simulink model "a"  (Simulink 7.0)
settings: Solver=FixedStepDiscrete  StartTime=0.0  StopTime=10.0  FixedStep=0.001  RelTol=1e-3
libraries: dsPICdrivers x6, fuzblock x1
settings Model: Creator=Administrator  LastModifiedBy=Administrator
settings OptimizationCC: OptimizeModelRefInitCode=on  LifeSpan=1
settings HardwareCC: ProdBitPerInt=16  ProdEndianess=LittleEndian  ProdWordSize=16  ProdHWDeviceType=16-bit Generic
settings RTWCC: SystemTargetFile=dspic.tlc  TemplateMakefile=dspic_pic30_gcc.tmf  PostCodeGenCommand=dsPIC_Compile()  Description=Embedded Target for Microchip dsPIC (real-time)  ProcessScript=dspic_make_rtw_hook
settings CodeAppCC: IgnoreCustomStorageClasses=off
settings STFCustomTargetCC: GenFloatMathFcnCalls=ANSI_C  ModelReferenceCompliant=off  IncludeMdlTerminateFcn=off  CombineOutputUpdateFcns=on  SuppressErrorStatus=on  ERTCustomFileBanners=on  SupportContinuousTime=off  SupportNonInlinedSFcns=off  SystemTargetFile=dspic.tlc
settings ERTTargetCC: GenFloatMathFcnCalls=ANSI_C  ModelReferenceCompliant=off  CompOptLevelCompliant=off  IncludeMdlTerminateFcn=off  SuppressErrorStatus=on  ModelStepFunctionPrototypeControlCompliant=off  ExtModeMexFile=noextcomm  InlinedParameterPlacement=NonHierarchical  ERTSrcFileBannerTemplate=dsPIC_code_template.cgt  ERTHdrFileBannerTemplate=dsPIC_code_template.cgt  ERTDataSrcFileTemplate=dsPIC_code_template.cgt  ERTDataHdrFileTemplate=dsPIC_code_template.cgt  ERTCustomFileTemplate=dsPIC_main.tlc
settings CustomProperty: DataType=string  Value=C:\PROGRA~1\MATLAB\R2007b\bin\win32\gmake

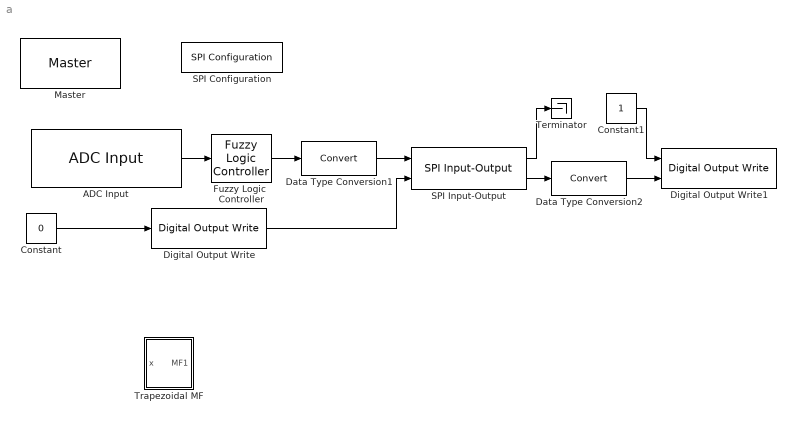
== system a ==
  ADC Input : dsPICdrivers/Peripheral I//O/ADC Input  Tag=dsPIC_ADC  Priority=5  ADC_TYPE=12 bits  ADC_MODE=Continuous sampling & get last channel value  NbrSampleStep=1  VoltRefpopup="AVdd  -  AVss"  OutFormatBitspopup=0000 dddd dddd dddd : Integer  InterruptPriority=6  ANCHANNELS=[8]  MaxName=ANmax = 4096  Rin=1e2  ADCS=6  SAMC=1  Temperature=25  DMAChannel=0  SampleTime=-1  Status="OK  |  Tsmp=7.000e-007 |  T/Channel=1.050e-005 |  Tall=1.050e-005"
  Constant : Constant  Value=0  OutDataTypeMode=boolean  OutDataType=sfix(16)  OutScaling=2^0
  Constant1 : Constant  OutDataTypeMode=boolean  OutDataType=sfix(16)  OutScaling=2^0
  Data Type Conversion1 : DataTypeConversion  OutDataTypeMode=uint16  OutDataType=sfix(16)  OutScaling=2^0
  Data Type Conversion2 : DataTypeConversion  OutDataTypeMode=boolean  OutDataType=sfix(16)  OutScaling=2^0
  Digital Output Write : dsPICdrivers/Digital I//O/Digital Output Write  Tag=dsPIC_Digital_Output  Priority=5  PORT=B  Pin=[2]  Simultaneous=off  OrderingInOutPopup=Output
  Digital Output Write1 : dsPICdrivers/Digital I//O/Digital Output Write  Tag=dsPIC_Digital_Output  Priority=5  PORT=B  Pin=[2]  Simultaneous=off  OrderingInOutPopup=Input
  Fuzzy Logic  Controller : fuzblock/Fuzzy Logic  Controller  SystemSampleTime=-1  fis=a1
  Master : dsPICdrivers/Master  Tag=dsPIC_MASTER  Priority=1  TimeStepType=Timer1  picType=30f6014  fcy=5e6  Quartz_33f=5e6  PLLActive_33f=off  fcyDesired_33f=0  tmr1="[1  4999  0]"  tmr1Info="Time Step : 0.001  ;   Error : 0%  PR1=4999"  tmr2345="[0  0  0  0]"  tmr2345cfg=[-1 -1 -1 -1]  IOautoConf=on  typePort="[ 0   0   0   0   0   0   0   0   0   0   0   0   0   0   0   0   0   0  10   0   0   0   0   0   8   0   0   0   0   0   0   0   0   0   0   0   0   0   0   0   0   0   0   0   0   0   0   0   0   0   0   0   0   0   0   0   0   0   0   0   0   0   0   0   0   0   0   0   0   0   0   0   0   0   0   0   0   0   0   0   0   0  14  15   0   0  16   0   0   0   0   0   0   0   0   0   0   0   0   0   0   0   0   0   0   0   0   0   0   0   0   0 ]"  TRIS="[ 65535  65531  65535  65535  65535  65535  65535 ]"  ADPCFG=4  MasterBusyPort=None  MasterOverloadPort=None  FOSC=LP  TempProtection_33f=TEMP_ON  FPBOR=PBOR_OFF  PWRT=PWRT_OFF  MCLR=MCLR_DIS  PowerSave=off
  SPI Configuration : dsPICdrivers/SPI PORT/SPI Configuration  Tag=dsPIC_config_SPI  Priority=2  ConfigurationTime=At boot time (only once)  OrderingInOutPopup=None  SampleTime=-1  Frame_Enable=0  Frame_Sync=None  SPI=1  MODE=SLAVE  USER_SCALER=20  StartEnable=Enable  SDO_EN=off  DATA_LENGTH=16 bits  SS_EN=off  SMP=End of bit  CKP=high  CKE=Idle to Active  Status="OK - Mode 1  -    Fsck= 250000Hz"
  SPI Input-Output : dsPICdrivers/SPI PORT/SPI Input-Output  Tag=dsPIC_SPI  SPI=1  INPUT=on  RESET_INPUT=off  OUTPUT=on  SPECIAL_SPI=Re-Enable Execute and Disable  DATA_LENGTH=16 bits  WAIT_INPUTDATA=on  OrderingInOutPopup=Input & Output  SampleTime=-1
  Terminator : Terminator
  Trapezoidal MF : Subsystem  AncestorBlock="fuzblock/Membership  Functions/Trapezoidal MF"  mask(trapmf){a=2, b=4, c=6, d=8}
      mask prompts: a "Left base point a:"; b "Left top point b:"; c "Right top point c:"; d "Right base point d:"
      mask help:
      | Trapezoidal membership function.
      |
      | The parameters a and d set the left and right "feet", or base points, of the trapezoid. The parameters b and c set the "shoulders", or top of the trapezoid.
      mask init:
      | x=-10:0.5:10;
      | params=[-8 -4 2 9];
      | y=trapmf(x,params);
      mask Help: eval('doc trapmf')
      mask Display: plot(x,y);
  wires:
  Digital Output Write/1 -> SPI Input-Output/2
  Constant/1 -> Digital Output Write/1
  Constant1/1 -> Digital Output Write1/1
  Data Type Conversion2/1 -> Digital Output Write1/2
  SPI Input-Output/2 -> Data Type Conversion2/1
  SPI Input-Output/1 -> Terminator/1
  ADC Input/1 -> Fuzzy Logic  Controller/1
  Fuzzy Logic  Controller/1 -> Data Type Conversion1/1
  Data Type Conversion1/1 -> SPI Input-Output/1

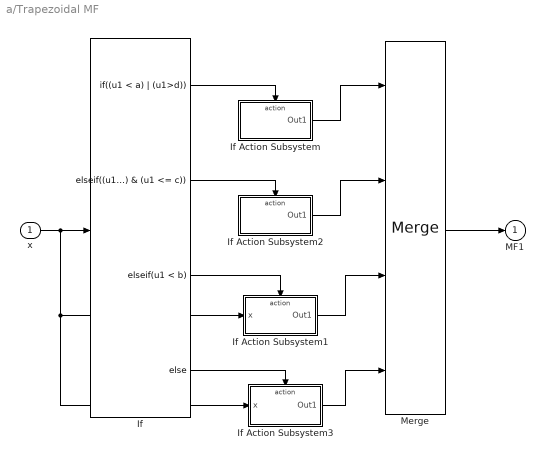
== system a/Trapezoidal MF ==
  x : Inport  OutDataType=sfix(16)  OutScaling=2^0
  If : If  IfExpression=(u1 < a) | (u1>d)  ElseIfExpressions=(u1 >= b) & (u1 <= c), u1 < b  ZeroCross=off
  If Action Subsystem : Subsystem  TreatAsAtomicUnit=on
  If Action Subsystem1 : Subsystem  TreatAsAtomicUnit=on
  If Action Subsystem2 : Subsystem  TreatAsAtomicUnit=on
  If Action Subsystem3 : Subsystem  TreatAsAtomicUnit=on
  Merge : Merge  Inputs=4
  MF1 : Outport  OutDataType=sfix(16)  OutScaling=2^0
  wires:
  If Action Subsystem3/1(Out1) -> Merge/4
  If Action Subsystem1/1(Out1) -> Merge/3
  If Action Subsystem2/1(Out1) -> Merge/2
  If/2 -> If Action Subsystem2/Action
  x/1 -> If Action Subsystem3/1(x), If Action Subsystem1/1(x), If/1
  If/3 -> If Action Subsystem1/Action
  If/4 -> If Action Subsystem3/Action
  If Action Subsystem/1(Out1) -> Merge/1
  Merge/1 -> MF1/1
  If/1 -> If Action Subsystem/Action

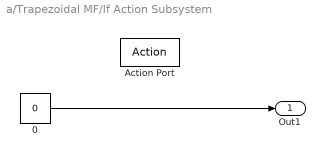
== system a/Trapezoidal MF/If Action Subsystem ==
  Action Port : ActionPort  ActionType=then
  0 : Constant  Value=0  OutDataTypeMode=double  OutDataType=sfix(16)  OutScaling=2^0
  Out1 : Outport  OutDataType=sfix(16)  OutScaling=2^0  InitialOutput=0
  wires:
  0/1 -> Out1/1

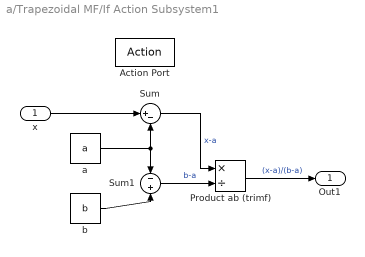
== system a/Trapezoidal MF/If Action Subsystem1 ==
  x : Inport  OutDataType=sfix(16)  OutScaling=2^0
  Action Port : ActionPort  ActionType=elseif
  Product ab (trimf) : Product  Inputs=*/  OutDataType=sfix(16)  OutScaling=2^0  SaturateOnIntegerOverflow=on  InputSameDT=on
  Sum : Sum  Inputs=|+-  OutDataType=sfix(16)  OutScaling=2^0  SaturateOnIntegerOverflow=on  InputSameDT=on
  Sum1 : Sum  Inputs=-+  OutDataType=sfix(16)  OutScaling=2^0  SaturateOnIntegerOverflow=on  InputSameDT=on
  a : Constant  Value=a  OutDataTypeMode=double  OutDataType=sfix(16)  OutScaling=2^0
  b : Constant  Value=b  OutDataTypeMode=double  OutDataType=sfix(16)  OutScaling=2^0
  Out1 : Outport  OutDataType=sfix(16)  OutScaling=2^0
  wires:
  Sum1/1 -> Product ab (trimf)/2  "b-a"
  Sum/1 -> Product ab (trimf)/1  "x-a"
  x/1 -> Sum/1
  b/1 -> Sum1/2
  a/1 -> Sum1/1, Sum/2
  Product ab (trimf)/1 -> Out1/1  "(x-a)/(b-a)"

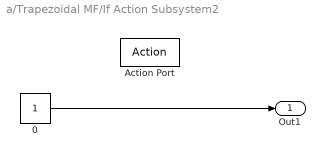
== system a/Trapezoidal MF/If Action Subsystem2 ==
  Action Port : ActionPort  ActionType=elseif
  0 : Constant  OutDataTypeMode=double  OutDataType=sfix(16)  OutScaling=2^0
  Out1 : Outport  OutDataType=sfix(16)  OutScaling=2^0  InitialOutput=0
  wires:
  0/1 -> Out1/1

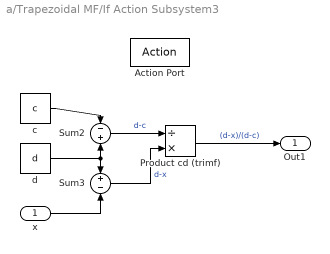
== system a/Trapezoidal MF/If Action Subsystem3 ==
  x : Inport  OutDataType=sfix(16)  OutScaling=2^0
  Action Port : ActionPort  ActionType=else
  Product cd (trimf) : Product  Inputs=/*  OutDataType=sfix(16)  OutScaling=2^0  SaturateOnIntegerOverflow=on  InputSameDT=on
  Sum2 : Sum  Inputs=-+  OutDataType=sfix(16)  OutScaling=2^0  SaturateOnIntegerOverflow=on  InputSameDT=on
  Sum3 : Sum  Inputs=+-  OutDataType=sfix(16)  OutScaling=2^0  SaturateOnIntegerOverflow=on  InputSameDT=on
  c : Constant  Value=c  OutDataTypeMode=double  OutDataType=sfix(16)  OutScaling=2^0
  d : Constant  Value=d  OutDataTypeMode=double  OutDataType=sfix(16)  OutScaling=2^0
  Out1 : Outport  OutDataType=sfix(16)  OutScaling=2^0
  wires:
  c/1 -> Sum2/1
  x/1 -> Sum3/2
  d/1 -> Sum3/1, Sum2/2
  Sum3/1 -> Product cd (trimf)/2  "d-x"
  Sum2/1 -> Product cd (trimf)/1  "d-c"
  Product cd (trimf)/1 -> Out1/1  "(d-x)/(d-c)"
